simulink model "ess_balancing_rig"  (R2025b)
settings: Solver=ode23t  StartTime=0.0  StopTime=10800  MaxStep=1  RelTol=1e-3
PreLoadFcn:
  | I_chg   = 1.25;               % charge current [A] (0.5C)
  | R_bleed = 47;                 % balancing (bleed) resistor [Ohm]
  | SOC0    = [0.80 0.75 0.75];   % initial SOC of Cell, Cell1, Cell2
libraries: nesl_utility x18, fl_lib x16, batteryecm_lib x3, BatteryBalancing x1
settings Model: Creator=Saquire  LastModifiedBy=Saquire
settings DataIOCC: SaveOutput=off

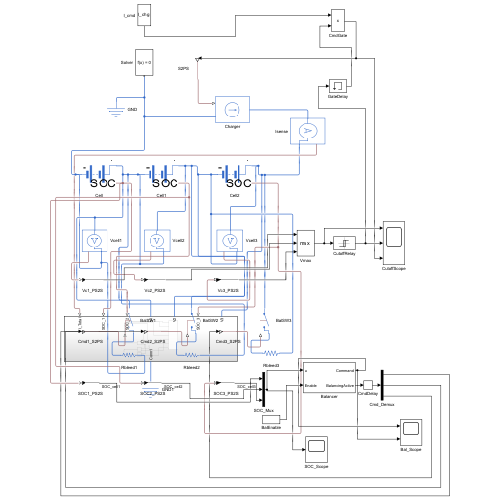
[thumbnail: Simulink's stored preview of the top-level diagram]
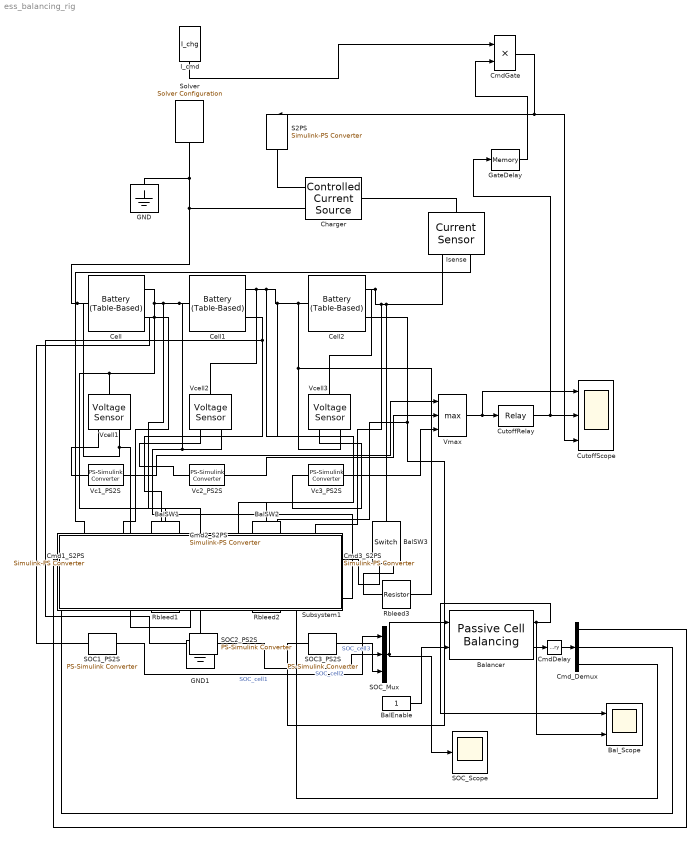
== system ess_balancing_rig ==
  BalEnable : Constant  OutDataTypeStr=boolean
  BalSW1 : fl_lib/Electrical/Electrical Elements/Switch  R_closed=0.01 Ohm  G_open=1e-8 1/Ohm  Threshold=0.5  i_specify=off  i_priority=None  i=0 A  i_nominal_specify=off  i_nominal_value=1  i_nominal_unit=A  v_specify=off  v_priority=None  v=0 V  v_nominal_specify=off  v_nominal_value=1  v_nominal_unit=V
  BalSW2 : fl_lib/Electrical/Electrical Elements/Switch  R_closed=0.01 Ohm  G_open=1e-8 1/Ohm  Threshold=0.5  i_specify=off  i_priority=None  i=0 A  i_nominal_specify=off  i_nominal_value=1  i_nominal_unit=A  v_specify=off  v_priority=None  v=0 V  v_nominal_specify=off  v_nominal_value=1  v_nominal_unit=V
  BalSW3 : fl_lib/Electrical/Electrical Elements/Switch  R_closed=0.01 Ohm  G_open=1e-8 1/Ohm  Threshold=0.5  i_specify=off  i_priority=None  i=0 A  i_nominal_specify=off  i_nominal_value=1  i_nominal_unit=A  v_specify=off  v_priority=None  v=0 V  v_nominal_specify=off  v_nominal_value=1  v_nominal_unit=V
  Bal_Scope : Scope  NumInputPorts=2
      settings: Title=Balancing commands / active  DataLoggingVariableName=balData
  Balancer : BatteryBalancing/Passive Cell Balancing  Threshold=0.01  HysteresisBand=0.005  Td_on=1  Td_off=1  Ts=1  dataType=double
      settings: LibrarySourceBlock=batt_sl_lib/Cell Balancing/Passive Cell Balancing
  Cell : batteryecm_lib/Battery (Table-Based)  SOC_vec=[0 .1 .2 .3 .4 .5 .6 .7 .8 .9 1]  T_dependence=simscape.enum.tablebattery.temperature_dependence.yes  prm_dir=simscape.enum.tablebattery.prm_dir.noCurrentDirectionality  T_vec=[278 293 313] K  V0_mat=[3.00 3.05 3.08;3.42 3.45 3.47;3.53 3.55 3.57;3.60 3.62 3.64;3.65 3.67 3.69;3.70 3.72 3.74;3.78 3.80 3.82;3.88 3.90 3.92;3.97 3.99 4.01;4.06 4.08 4.10;4.16 4.18 4.19] V  V0_vec=[3.5057, 3.566, 3.6337, 3.7127, 3.9259, 4.0777, 4.1928] V  V_range=[2.5 4.3] V  R0_mat=[.070 .045 .035;.055 .036 .028;.050 .033 .026;.048 .032 .025;.046 .031 .024;.045 .030 .024;.045 .030 .024;.045 .030 .024;.046 .031 .025;.047 .031 .025;.048 .032 .026] Ohm  R0_vec=[.0085, .0085, .0087, .0082, .0083, .0085, .0085] Ohm  R0_dis_mat=[.0117, .0085, .009; .011, .0085, .009; .0114, .0087, .0092; .0107, .0082, .0088; .0107, .0083, .0091; .0113, .0085, .0089; .0116, .0085, .0089] Ohm  R0_dis_vec=[.0085, .0085, .0087, .0082, .0083, .0085, .0085] Ohm  R0_ch_mat=[.0117, .0085, .009; .011, .0085, .009; .0114, .0087, .0092; .0107, .0082, .0088; .0107, .0083, .0091; .0113, .0085, .0089; .0116, .0085, .0089] Ohm  R0_ch_vec=[.0085, .0085, .0087, .0082, .0083, .0085, .0085] Ohm  AH=2.5 A*hr  prm_leak=simscape.enum.tablebattery.prm_leak.disabled  Rleak_vec=[8000, 7000, 6000] Ohm  Rleak=7e3 Ohm  extrapolation_option=simscape.enum.extrapolation.nearest  SOC_port=simscape.enum.tablebattery.enable.yes  prm_dyn=simscape.enum.tablebattery.prm_dyn.off  R1_mat=[.0109, .0029, .0013; .0069, .0024, .0012; .0047, .0026, .0013; .0034, .0016, .001; .0033, .0023, .0014; .0033, .0018, .0011; .0028, .0017, .0011] Ohm  R1_vec=[.0029, .0024, .0026, .0016, .0023, .0018, .0017] Ohm  tau1_mat=[20, 36, 39; 31, 45, 39; 109, 105, 61; 36, 29, 26; 59, 77, 67; 40, 33, 29; 25, 39, 33] s  tau1_vec=[36, 45, 105, 29, 77, 33, 39] s  R2_mat=[.0109, .0029, .0013; .0069, .0024, .0012; .0047, .0026, .0013; .0034, .0016, .001; .0033, .0023, .0014; .0033, .0018, .0011; .0028, .0017, .0011] Ohm  R2_vec=[.0029, .0024, .0026, .0016, .0023, .0018, .0017] Ohm  tau2_mat=[20, 36, 39; 31, 45, 39; 109, 105, 61; 36, 29, 26; 59, 77, 67; 40, 33, 29; 25, 39, 33] s  tau2_vec=[36, 45, 105, 29, 77, 33, 39] s  R3_mat=[.0109, .0029, .0013; .0069, .0024, .0012; .0047, .0026, .0013; .0034, .0016, .001; .0033, .0023, .0014; .0033, .0018, .0011; .0028, .0017, .0011] Ohm  R3_vec=[.0029, .0024, .0026, .0016, .0023, .0018, .0017] Ohm  tau3_mat=[20, 36, 39; 31, 45, 39; 109, 105, 61; 36, 29, 26; 59, 77, 67; 40, 33, 29; 25, 39, 33] s  tau3_vec=[36, 45, 105, 29, 77, 33, 39] s  R4_mat=[.0109, .0029, .0013; .0069, .0024, .0012; .0047, .0026, .0013; .0034, .0016, .001; .0033, .0023, .0014; .0033, .0018, .0011; .0028, .0017, .0011] Ohm  R4_vec=[.0029, .0024, .0026, .0016, .0023, .0018, .0017] Ohm  tau4_mat=[20, 36, 39; 31, 45, 39; 109, 105, 61; 36, 29, 26; 59, 77, 67; 40, 33, 29; 25, 39, 33] s  tau4_vec=[36, 45, 105, 29, 77, 33, 39] s  R5_mat=[.0109, .0029, .0013; .0069, .0024, .0012; .0047, .0026, .0013; .0034, .0016, .001; .0033, .0023, .0014; .0033, .0018, .0011; .0028, .0017, .0011] Ohm  R5_vec=[.0029, .0024, .0026, .0016, .0023, .0018, .0017] Ohm  tau5_mat=[20, 36, 39; 31, 45, 39; 109, 105, 61; 36, 29, 26; 59, 77, 67; 40, 33, 29; 25, 39, 33] s  tau5_vec=[36, 45, 105, 29, 77, 33, 39] s  prm_fade=simscape.enum.tablebattery.prm_fade.disabled  N0=100  dV0=0  dR0=0  dAH=0  dRleak=0  dR1=0  dR2=0  dR3=0  dR4=0  dR5=0  N0vec=[0, 100, 200, 300]  Tfadevec=[298.15, 323.15] K  dV0vec=[0, 0, 0, 0]  dR0vec=[0, 0, 0, 0]  dAHvec=[0, 0, 0, 0]  dRleakvec=[0, 0, 0, 0]  dR1vec=[0, 0, 0, 0]  dR2vec=[0, 0, 0, 0]  dR3vec=[0, 0, 0, 0]  dR4vec=[0, 0, 0, 0]  dR5vec=[0, 0, 0, 0]  dV0mat=[0, 0; 0, 0; 0, 0; 0, 0]  dR0mat=[0, 0; 0, 0; 0, 0; 0, 0]  dAHmat=[0, 0; 0, 0; 0, 0; 0, 0]  dRleakmat=[0, 0; 0, 0; 0, 0; 0, 0]  dR1mat=[0, 0; 0, 0; 0, 0; 0, 0]  dR2mat=[0, 0; 0, 0; 0, 0; 0, 0]  dR3mat=[0, 0; 0, 0; 0, 0; 0, 0]  dR4mat=[0, 0; 0, 0; 0, 0; 0, 0]  dR5mat=[0, 0; 0, 0; 0, 0; 0, 0]  prm_age_modeling=simscape.enum.tablebattery.prm_age_modeling.equation  storage_dt_age_vec=[0] d  storage_T_age_vec=[273] K  prm_age_OCV=simscape.enum.tablebattery.prm_age_OCV.OCV  OCV_age=0.9  SOC_age=0.6  prm_age_resistance=simscape.enum.tablebattery.prm_age.disabled  OCV_scaling_age_resistance=2.2134e6  OCV_offset_age_resistance=1.632e6  temp_exp_age_resistance=0.515833569 V  t_exp_age_resistance=0.75  T_age_vec_resistance=[273.15, 298.15, 323.15] K  dt_age_vec_resistance=[0, 90, 180, 270] d  dR0_age_vec=[0, 0, 0]  t_meas_dR0_age=100 d  dR0_age_mat=[0, 0, 0; 0, 0, 0; 0, 0, 0; 0, 0, 0]  prm_age_capacity=simscape.enum.tablebattery.prm_age.disabled  OCV_scaling_age_capacity=1.5097e07  OCV_offset_age_capacity=8.3625e06  temp_exp_age_capacity=0.6011 V  t_exp_age_capacity=0.75  T_age_vec_capacity=[273.15, 298.15, 323.15] K  dt_age_vec_capacity=[0, 90, 180, 270] d  dAH_age_vec=[0, 0, 0]  t_meas_dAH_age=100 d  dAH_age_mat=[0, 0, 0; 0, 0, 0; 0, 0, 0; 0, 0, 0]  thermal_port=simscape.enum.thermaleffects.omit  temperature=298.15 K  thermal_mass=100 J/K  i_specify=off  i_priority=None  i=0 A  i_nominal_specify=off  i_nominal_value=1  i_nominal_unit=A  v_specify=off  v_priority=None  v=0 V  v_nominal_specify=off  v_nominal_value=1  v_nominal_unit=V  stateOfCharge_specify=on  stateOfCharge_priority=High  stateOfCharge=SOC0(1)  stateOfCharge_nominal_specify=off  stateOfCharge_nominal_value=1  stateOfCharge_nominal_unit=1  num_cycles_specify=off  num_cycles_priority=High  num_cycles=0  num_cycles_nominal_specify=off  num_cycles_nominal_value=1  num_cycles_nominal_unit=1  cell_temperature_specify=off  cell_temperature_priority=High  cell_temperature=298.15 K  cell_temperature_nominal_specify=off  cell_temperature_nominal_value=1  cell_temperature_nominal_unit=K
      settings: InternalSimscapePortConfiguration="{\"Bottom\":[],\"Left\":[{\"id\":\"p\",\"label\":\"+\",\"type\":\"foundation.electrical.electrical\"},{\"id\":\"soc\",\"label\":\"SOC\",\"type\":\"output\"}],\"Right\":[{\"id\":\"n\",\"label\":\"-\",\"type\":\"foundation.electrical.electrical\"}],\"Top\":[]}"
  Cell1 : batteryecm_lib/Battery (Table-Based)  SOC_vec=[0 .1 .2 .3 .4 .5 .6 .7 .8 .9 1]  T_dependence=simscape.enum.tablebattery.temperature_dependence.yes  prm_dir=simscape.enum.tablebattery.prm_dir.noCurrentDirectionality  T_vec=[278 293 313] K  V0_mat=[3.00 3.05 3.08;3.42 3.45 3.47;3.53 3.55 3.57;3.60 3.62 3.64;3.65 3.67 3.69;3.70 3.72 3.74;3.78 3.80 3.82;3.88 3.90 3.92;3.97 3.99 4.01;4.06 4.08 4.10;4.16 4.18 4.19] V  V0_vec=[3.5057, 3.566, 3.6337, 3.7127, 3.9259, 4.0777, 4.1928] V  V_range=[2.5 4.3] V  R0_mat=[.070 .045 .035;.055 .036 .028;.050 .033 .026;.048 .032 .025;.046 .031 .024;.045 .030 .024;.045 .030 .024;.045 .030 .024;.046 .031 .025;.047 .031 .025;.048 .032 .026] Ohm  R0_vec=[.0085, .0085, .0087, .0082, .0083, .0085, .0085] Ohm  R0_dis_mat=[.0117, .0085, .009; .011, .0085, .009; .0114, .0087, .0092; .0107, .0082, .0088; .0107, .0083, .0091; .0113, .0085, .0089; .0116, .0085, .0089] Ohm  R0_dis_vec=[.0085, .0085, .0087, .0082, .0083, .0085, .0085] Ohm  R0_ch_mat=[.0117, .0085, .009; .011, .0085, .009; .0114, .0087, .0092; .0107, .0082, .0088; .0107, .0083, .0091; .0113, .0085, .0089; .0116, .0085, .0089] Ohm  R0_ch_vec=[.0085, .0085, .0087, .0082, .0083, .0085, .0085] Ohm  AH=2.5 A*hr  prm_leak=simscape.enum.tablebattery.prm_leak.disabled  Rleak_vec=[8000, 7000, 6000] Ohm  Rleak=7e3 Ohm  extrapolation_option=simscape.enum.extrapolation.nearest  SOC_port=simscape.enum.tablebattery.enable.yes  prm_dyn=simscape.enum.tablebattery.prm_dyn.off  R1_mat=[.0109, .0029, .0013; .0069, .0024, .0012; .0047, .0026, .0013; .0034, .0016, .001; .0033, .0023, .0014; .0033, .0018, .0011; .0028, .0017, .0011] Ohm  R1_vec=[.0029, .0024, .0026, .0016, .0023, .0018, .0017] Ohm  tau1_mat=[20, 36, 39; 31, 45, 39; 109, 105, 61; 36, 29, 26; 59, 77, 67; 40, 33, 29; 25, 39, 33] s  tau1_vec=[36, 45, 105, 29, 77, 33, 39] s  R2_mat=[.0109, .0029, .0013; .0069, .0024, .0012; .0047, .0026, .0013; .0034, .0016, .001; .0033, .0023, .0014; .0033, .0018, .0011; .0028, .0017, .0011] Ohm  R2_vec=[.0029, .0024, .0026, .0016, .0023, .0018, .0017] Ohm  tau2_mat=[20, 36, 39; 31, 45, 39; 109, 105, 61; 36, 29, 26; 59, 77, 67; 40, 33, 29; 25, 39, 33] s  tau2_vec=[36, 45, 105, 29, 77, 33, 39] s  R3_mat=[.0109, .0029, .0013; .0069, .0024, .0012; .0047, .0026, .0013; .0034, .0016, .001; .0033, .0023, .0014; .0033, .0018, .0011; .0028, .0017, .0011] Ohm  R3_vec=[.0029, .0024, .0026, .0016, .0023, .0018, .0017] Ohm  tau3_mat=[20, 36, 39; 31, 45, 39; 109, 105, 61; 36, 29, 26; 59, 77, 67; 40, 33, 29; 25, 39, 33] s  tau3_vec=[36, 45, 105, 29, 77, 33, 39] s  R4_mat=[.0109, .0029, .0013; .0069, .0024, .0012; .0047, .0026, .0013; .0034, .0016, .001; .0033, .0023, .0014; .0033, .0018, .0011; .0028, .0017, .0011] Ohm  R4_vec=[.0029, .0024, .0026, .0016, .0023, .0018, .0017] Ohm  tau4_mat=[20, 36, 39; 31, 45, 39; 109, 105, 61; 36, 29, 26; 59, 77, 67; 40, 33, 29; 25, 39, 33] s  tau4_vec=[36, 45, 105, 29, 77, 33, 39] s  R5_mat=[.0109, .0029, .0013; .0069, .0024, .0012; .0047, .0026, .0013; .0034, .0016, .001; .0033, .0023, .0014; .0033, .0018, .0011; .0028, .0017, .0011] Ohm  R5_vec=[.0029, .0024, .0026, .0016, .0023, .0018, .0017] Ohm  tau5_mat=[20, 36, 39; 31, 45, 39; 109, 105, 61; 36, 29, 26; 59, 77, 67; 40, 33, 29; 25, 39, 33] s  tau5_vec=[36, 45, 105, 29, 77, 33, 39] s  prm_fade=simscape.enum.tablebattery.prm_fade.disabled  N0=100  dV0=0  dR0=0  dAH=0  dRleak=0  dR1=0  dR2=0  dR3=0  dR4=0  dR5=0  N0vec=[0, 100, 200, 300]  Tfadevec=[298.15, 323.15] K  dV0vec=[0, 0, 0, 0]  dR0vec=[0, 0, 0, 0]  dAHvec=[0, 0, 0, 0]  dRleakvec=[0, 0, 0, 0]  dR1vec=[0, 0, 0, 0]  dR2vec=[0, 0, 0, 0]  dR3vec=[0, 0, 0, 0]  dR4vec=[0, 0, 0, 0]  dR5vec=[0, 0, 0, 0]  dV0mat=[0, 0; 0, 0; 0, 0; 0, 0]  dR0mat=[0, 0; 0, 0; 0, 0; 0, 0]  dAHmat=[0, 0; 0, 0; 0, 0; 0, 0]  dRleakmat=[0, 0; 0, 0; 0, 0; 0, 0]  dR1mat=[0, 0; 0, 0; 0, 0; 0, 0]  dR2mat=[0, 0; 0, 0; 0, 0; 0, 0]  dR3mat=[0, 0; 0, 0; 0, 0; 0, 0]  dR4mat=[0, 0; 0, 0; 0, 0; 0, 0]  dR5mat=[0, 0; 0, 0; 0, 0; 0, 0]  prm_age_modeling=simscape.enum.tablebattery.prm_age_modeling.equation  storage_dt_age_vec=[0] d  storage_T_age_vec=[273] K  prm_age_OCV=simscape.enum.tablebattery.prm_age_OCV.OCV  OCV_age=0.9  SOC_age=0.6  prm_age_resistance=simscape.enum.tablebattery.prm_age.disabled  OCV_scaling_age_resistance=2.2134e6  OCV_offset_age_resistance=1.632e6  temp_exp_age_resistance=0.515833569 V  t_exp_age_resistance=0.75  T_age_vec_resistance=[273.15, 298.15, 323.15] K  dt_age_vec_resistance=[0, 90, 180, 270] d  dR0_age_vec=[0, 0, 0]  t_meas_dR0_age=100 d  dR0_age_mat=[0, 0, 0; 0, 0, 0; 0, 0, 0; 0, 0, 0]  prm_age_capacity=simscape.enum.tablebattery.prm_age.disabled  OCV_scaling_age_capacity=1.5097e07  OCV_offset_age_capacity=8.3625e06  temp_exp_age_capacity=0.6011 V  t_exp_age_capacity=0.75  T_age_vec_capacity=[273.15, 298.15, 323.15] K  dt_age_vec_capacity=[0, 90, 180, 270] d  dAH_age_vec=[0, 0, 0]  t_meas_dAH_age=100 d  dAH_age_mat=[0, 0, 0; 0, 0, 0; 0, 0, 0; 0, 0, 0]  thermal_port=simscape.enum.thermaleffects.omit  temperature=298.15 K  thermal_mass=100 J/K  i_specify=off  i_priority=None  i=0 A  i_nominal_specify=off  i_nominal_value=1  i_nominal_unit=A  v_specify=off  v_priority=None  v=0 V  v_nominal_specify=off  v_nominal_value=1  v_nominal_unit=V  stateOfCharge_specify=on  stateOfCharge_priority=High  stateOfCharge=SOC0(2)  stateOfCharge_nominal_specify=off  stateOfCharge_nominal_value=0.6  stateOfCharge_nominal_unit=1  num_cycles_specify=off  num_cycles_priority=High  num_cycles=0  num_cycles_nominal_specify=off  num_cycles_nominal_value=1  num_cycles_nominal_unit=1  cell_temperature_specify=off  cell_temperature_priority=High  cell_temperature=298.15 K  cell_temperature_nominal_specify=off  cell_temperature_nominal_value=1  cell_temperature_nominal_unit=K
      settings: InternalSimscapePortConfiguration="{\"Bottom\":[],\"Left\":[{\"id\":\"p\",\"label\":\"+\",\"type\":\"foundation.electrical.electrical\"},{\"id\":\"soc\",\"label\":\"SOC\",\"type\":\"output\"}],\"Right\":[{\"id\":\"n\",\"label\":\"-\",\"type\":\"foundation.electrical.electrical\"}],\"Top\":[]}"
  Cell2 : batteryecm_lib/Battery (Table-Based)  SOC_vec=[0 .1 .2 .3 .4 .5 .6 .7 .8 .9 1]  T_dependence=simscape.enum.tablebattery.temperature_dependence.yes  prm_dir=simscape.enum.tablebattery.prm_dir.noCurrentDirectionality  T_vec=[278 293 313] K  V0_mat=[3.00 3.05 3.08;3.42 3.45 3.47;3.53 3.55 3.57;3.60 3.62 3.64;3.65 3.67 3.69;3.70 3.72 3.74;3.78 3.80 3.82;3.88 3.90 3.92;3.97 3.99 4.01;4.06 4.08 4.10;4.16 4.18 4.19] V  V0_vec=[3.5057, 3.566, 3.6337, 3.7127, 3.9259, 4.0777, 4.1928] V  V_range=[2.5 4.3] V  R0_mat=[.070 .045 .035;.055 .036 .028;.050 .033 .026;.048 .032 .025;.046 .031 .024;.045 .030 .024;.045 .030 .024;.045 .030 .024;.046 .031 .025;.047 .031 .025;.048 .032 .026] Ohm  R0_vec=[.0085, .0085, .0087, .0082, .0083, .0085, .0085] Ohm  R0_dis_mat=[.0117, .0085, .009; .011, .0085, .009; .0114, .0087, .0092; .0107, .0082, .0088; .0107, .0083, .0091; .0113, .0085, .0089; .0116, .0085, .0089] Ohm  R0_dis_vec=[.0085, .0085, .0087, .0082, .0083, .0085, .0085] Ohm  R0_ch_mat=[.0117, .0085, .009; .011, .0085, .009; .0114, .0087, .0092; .0107, .0082, .0088; .0107, .0083, .0091; .0113, .0085, .0089; .0116, .0085, .0089] Ohm  R0_ch_vec=[.0085, .0085, .0087, .0082, .0083, .0085, .0085] Ohm  AH=2.5 A*hr  prm_leak=simscape.enum.tablebattery.prm_leak.disabled  Rleak_vec=[8000, 7000, 6000] Ohm  Rleak=7e3 Ohm  extrapolation_option=simscape.enum.extrapolation.nearest  SOC_port=simscape.enum.tablebattery.enable.yes  prm_dyn=simscape.enum.tablebattery.prm_dyn.off  R1_mat=[.0109, .0029, .0013; .0069, .0024, .0012; .0047, .0026, .0013; .0034, .0016, .001; .0033, .0023, .0014; .0033, .0018, .0011; .0028, .0017, .0011] Ohm  R1_vec=[.0029, .0024, .0026, .0016, .0023, .0018, .0017] Ohm  tau1_mat=[20, 36, 39; 31, 45, 39; 109, 105, 61; 36, 29, 26; 59, 77, 67; 40, 33, 29; 25, 39, 33] s  tau1_vec=[36, 45, 105, 29, 77, 33, 39] s  R2_mat=[.0109, .0029, .0013; .0069, .0024, .0012; .0047, .0026, .0013; .0034, .0016, .001; .0033, .0023, .0014; .0033, .0018, .0011; .0028, .0017, .0011] Ohm  R2_vec=[.0029, .0024, .0026, .0016, .0023, .0018, .0017] Ohm  tau2_mat=[20, 36, 39; 31, 45, 39; 109, 105, 61; 36, 29, 26; 59, 77, 67; 40, 33, 29; 25, 39, 33] s  tau2_vec=[36, 45, 105, 29, 77, 33, 39] s  R3_mat=[.0109, .0029, .0013; .0069, .0024, .0012; .0047, .0026, .0013; .0034, .0016, .001; .0033, .0023, .0014; .0033, .0018, .0011; .0028, .0017, .0011] Ohm  R3_vec=[.0029, .0024, .0026, .0016, .0023, .0018, .0017] Ohm  tau3_mat=[20, 36, 39; 31, 45, 39; 109, 105, 61; 36, 29, 26; 59, 77, 67; 40, 33, 29; 25, 39, 33] s  tau3_vec=[36, 45, 105, 29, 77, 33, 39] s  R4_mat=[.0109, .0029, .0013; .0069, .0024, .0012; .0047, .0026, .0013; .0034, .0016, .001; .0033, .0023, .0014; .0033, .0018, .0011; .0028, .0017, .0011] Ohm  R4_vec=[.0029, .0024, .0026, .0016, .0023, .0018, .0017] Ohm  tau4_mat=[20, 36, 39; 31, 45, 39; 109, 105, 61; 36, 29, 26; 59, 77, 67; 40, 33, 29; 25, 39, 33] s  tau4_vec=[36, 45, 105, 29, 77, 33, 39] s  R5_mat=[.0109, .0029, .0013; .0069, .0024, .0012; .0047, .0026, .0013; .0034, .0016, .001; .0033, .0023, .0014; .0033, .0018, .0011; .0028, .0017, .0011] Ohm  R5_vec=[.0029, .0024, .0026, .0016, .0023, .0018, .0017] Ohm  tau5_mat=[20, 36, 39; 31, 45, 39; 109, 105, 61; 36, 29, 26; 59, 77, 67; 40, 33, 29; 25, 39, 33] s  tau5_vec=[36, 45, 105, 29, 77, 33, 39] s  prm_fade=simscape.enum.tablebattery.prm_fade.disabled  N0=100  dV0=0  dR0=0  dAH=0  dRleak=0  dR1=0  dR2=0  dR3=0  dR4=0  dR5=0  N0vec=[0, 100, 200, 300]  Tfadevec=[298.15, 323.15] K  dV0vec=[0, 0, 0, 0]  dR0vec=[0, 0, 0, 0]  dAHvec=[0, 0, 0, 0]  dRleakvec=[0, 0, 0, 0]  dR1vec=[0, 0, 0, 0]  dR2vec=[0, 0, 0, 0]  dR3vec=[0, 0, 0, 0]  dR4vec=[0, 0, 0, 0]  dR5vec=[0, 0, 0, 0]  dV0mat=[0, 0; 0, 0; 0, 0; 0, 0]  dR0mat=[0, 0; 0, 0; 0, 0; 0, 0]  dAHmat=[0, 0; 0, 0; 0, 0; 0, 0]  dRleakmat=[0, 0; 0, 0; 0, 0; 0, 0]  dR1mat=[0, 0; 0, 0; 0, 0; 0, 0]  dR2mat=[0, 0; 0, 0; 0, 0; 0, 0]  dR3mat=[0, 0; 0, 0; 0, 0; 0, 0]  dR4mat=[0, 0; 0, 0; 0, 0; 0, 0]  dR5mat=[0, 0; 0, 0; 0, 0; 0, 0]  prm_age_modeling=simscape.enum.tablebattery.prm_age_modeling.equation  storage_dt_age_vec=[0] d  storage_T_age_vec=[273] K  prm_age_OCV=simscape.enum.tablebattery.prm_age_OCV.OCV  OCV_age=0.9  SOC_age=0.6  prm_age_resistance=simscape.enum.tablebattery.prm_age.disabled  OCV_scaling_age_resistance=2.2134e6  OCV_offset_age_resistance=1.632e6  temp_exp_age_resistance=0.515833569 V  t_exp_age_resistance=0.75  T_age_vec_resistance=[273.15, 298.15, 323.15] K  dt_age_vec_resistance=[0, 90, 180, 270] d  dR0_age_vec=[0, 0, 0]  t_meas_dR0_age=100 d  dR0_age_mat=[0, 0, 0; 0, 0, 0; 0, 0, 0; 0, 0, 0]  prm_age_capacity=simscape.enum.tablebattery.prm_age.disabled  OCV_scaling_age_capacity=1.5097e07  OCV_offset_age_capacity=8.3625e06  temp_exp_age_capacity=0.6011 V  t_exp_age_capacity=0.75  T_age_vec_capacity=[273.15, 298.15, 323.15] K  dt_age_vec_capacity=[0, 90, 180, 270] d  dAH_age_vec=[0, 0, 0]  t_meas_dAH_age=100 d  dAH_age_mat=[0, 0, 0; 0, 0, 0; 0, 0, 0; 0, 0, 0]  thermal_port=simscape.enum.thermaleffects.omit  temperature=298.15 K  thermal_mass=100 J/K  i_specify=off  i_priority=None  i=0 A  i_nominal_specify=off  i_nominal_value=1  i_nominal_unit=A  v_specify=off  v_priority=None  v=0 V  v_nominal_specify=off  v_nominal_value=1  v_nominal_unit=V  stateOfCharge_specify=on  stateOfCharge_priority=High  stateOfCharge=SOC0(3)  stateOfCharge_nominal_specify=off  stateOfCharge_nominal_value=0.6  stateOfCharge_nominal_unit=1  num_cycles_specify=off  num_cycles_priority=High  num_cycles=0  num_cycles_nominal_specify=off  num_cycles_nominal_value=1  num_cycles_nominal_unit=1  cell_temperature_specify=off  cell_temperature_priority=High  cell_temperature=298.15 K  cell_temperature_nominal_specify=off  cell_temperature_nominal_value=1  cell_temperature_nominal_unit=K
      settings: InternalSimscapePortConfiguration="{\"Bottom\":[],\"Left\":[{\"id\":\"p\",\"label\":\"+\",\"type\":\"foundation.electrical.electrical\"},{\"id\":\"soc\",\"label\":\"SOC\",\"type\":\"output\"}],\"Right\":[{\"id\":\"n\",\"label\":\"-\",\"type\":\"foundation.electrical.electrical\"}],\"Top\":[]}"
  Charger : fl_lib/Electrical/Electrical Sources/Controlled Current Source
  Cmd1_S2PS : nesl_utility/Simulink-PS Converter  PhysicalDomain=network_engine_domain  SubClassName=ps_input  LeftPortType=input  RightPortType=output  PseudoPeriodic=off  Frequencies=[]  NoiseDistribution=none  NoiseParameters=[]  Unit=1  AffineConversion=off  FilteringAndDerivatives=provide  SimscapeFilterOrder=1  InputFilterTimeConstant=0.001  UdotUserProvided=0
  Cmd2_S2PS : nesl_utility/Simulink-PS Converter  PhysicalDomain=network_engine_domain  SubClassName=ps_input  LeftPortType=input  RightPortType=output  PseudoPeriodic=off  Frequencies=[]  NoiseDistribution=none  NoiseParameters=[]  Unit=1  AffineConversion=off  FilteringAndDerivatives=provide  SimscapeFilterOrder=1  InputFilterTimeConstant=0.001  UdotUserProvided=0
  Cmd3_S2PS : nesl_utility/Simulink-PS Converter  PhysicalDomain=network_engine_domain  SubClassName=ps_input  LeftPortType=input  RightPortType=output  PseudoPeriodic=off  Frequencies=[]  NoiseDistribution=none  NoiseParameters=[]  Unit=1  AffineConversion=off  FilteringAndDerivatives=provide  SimscapeFilterOrder=1  InputFilterTimeConstant=0.001  UdotUserProvided=0
  CmdDelay : Memory
  CmdGate : Product
  Cmd_Demux : Demux  Outputs=3
  CutoffRelay : Relay  OnSwitchValue=4.2  OffSwitchValue=4.15  OnOutputValue=0  OffOutputValue=1
  CutoffScope : Scope  NumInputPorts=3
      settings: ActiveDisplayYMinimum=-9.1766114496806388  ActiveDisplayYMaximum=10.823388550319361  DataLoggingVariableName=cutoffData
  GND : fl_lib/Electrical/Electrical Elements/Electrical Reference
  GND1 : fl_lib/Electrical/Electrical Elements/Electrical Reference
  GateDelay : Memory  InitialCondition=1
  I_cmd : Constant  Value=I_chg
  Isense : fl_lib/Electrical/Electrical Sensors/Current Sensor
  Rbleed1 : fl_lib/Electrical/Electrical Elements/Resistor  R=R_bleed Ohm  i_specify=off  i_priority=None  i=0 A  i_nominal_specify=off  i_nominal_value=1  i_nominal_unit=A  v_specify=off  v_priority=None  v=0 V  v_nominal_specify=off  v_nominal_value=1  v_nominal_unit=V
  Rbleed2 : fl_lib/Electrical/Electrical Elements/Resistor  R=R_bleed Ohm  i_specify=off  i_priority=None  i=0 A  i_nominal_specify=off  i_nominal_value=1  i_nominal_unit=A  v_specify=off  v_priority=None  v=0 V  v_nominal_specify=off  v_nominal_value=1  v_nominal_unit=V
  Rbleed3 : fl_lib/Electrical/Electrical Elements/Resistor  R=R_bleed Ohm  i_specify=off  i_priority=None  i=0 A  i_nominal_specify=off  i_nominal_value=1  i_nominal_unit=A  v_specify=off  v_priority=None  v=0 V  v_nominal_specify=off  v_nominal_value=1  v_nominal_unit=V
  S2PS : nesl_utility/Simulink-PS Converter  PhysicalDomain=network_engine_domain  SubClassName=ps_input  LeftPortType=input  RightPortType=output  PseudoPeriodic=off  Frequencies=[]  NoiseDistribution=none  NoiseParameters=[]  Unit=1  AffineConversion=off  FilteringAndDerivatives=provide  SimscapeFilterOrder=1  InputFilterTimeConstant=0.001  UdotUserProvided=0
  SOC1_PS2S : nesl_utility/PS-Simulink Converter  PhysicalDomain=network_engine_domain  SubClassName=ps_output  LeftPortType=input  RightPortType=output  PseudoPeriodic=off  Frequencies=[]  VectorFormat=inherit  Unit=inherit  AffineConversion=off
  SOC2_PS2S : nesl_utility/PS-Simulink Converter  PhysicalDomain=network_engine_domain  SubClassName=ps_output  LeftPortType=input  RightPortType=output  PseudoPeriodic=off  Frequencies=[]  VectorFormat=inherit  Unit=inherit  AffineConversion=off
  SOC3_PS2S : nesl_utility/PS-Simulink Converter  PhysicalDomain=network_engine_domain  SubClassName=ps_output  LeftPortType=input  RightPortType=output  PseudoPeriodic=off  Frequencies=[]  VectorFormat=inherit  Unit=inherit  AffineConversion=off
  SOC_Mux : Mux  Inputs=3
  SOC_Scope : Scope
      settings: Title=Cell SOCs  ActiveDisplayYMinimum=0.7  ActiveDisplayYMaximum=1  YLabel=SOC  DataLoggingVariableName=socData
  Solver : nesl_utility/Solver Configuration  PhysicalDomain=network_engine_domain  SubClassName=solver  LeftPortType=input  RightPortType=generic  Tones=[]  Harmonics=[]  SimulateNoise=off  Profile=off  UseLocalSampling=off  EnableSwitchedLinearOptims=on  FrequencyDomain=off  UseCCode=off  RelTol=0.001  AbsTol=0.001  MinStep=1e-09  ToWorkspace=off  RevertToSquareIcSolve=off  NumHomotopyIterations=100  PhasorMode=off  PhasorModeNumHarmonics=1  ConsistencySolver=NEWTON_XTOL_AFTER_FTOL  IndexReductionMethod=DerivativeReplacement  DoDC=off  ResidualTolerance=1e-09  ConsistencyTolSource=GLOBAL  ConsistencyAbsTol=0.001  ConsistencyRelTol=0.001  ConsistencyTolFactor=0.001  UseLocalSolver=off  LocalSolverChoice=NE_BACKWARD_EULER_ADVANCER  ResolveIndetEquations=on  FunctionEvalNumThread=1  LocalSolverSampleTime=0.001  DoFixedCost=off  MaxNonlinIter=3  MaxModeIter=2  ComputeImpulses=off  ImpulseIterations=2  LinearAlgebra=auto  LinearAlgebraNumThread=0  EquationFormulation=NE_TIME_EF  DelaysMemoryBudget=1024  AutomaticFiltering=on  FilteringTimeConstant=0.001  PartitionStorageMethod=AS_NEEDED  PartitionMemoryBudget=1024  PartitionMethod=ROBUST  MultibodyUseLocalSolver=off  MultibodyLocalSolverChoice=ODE1  MultibodyLocalSolverSampleTime=0.001
  Subsystem1 : Subsystem
  Vc1_PS2S : nesl_utility/PS-Simulink Converter  PhysicalDomain=network_engine_domain  SubClassName=ps_output  LeftPortType=input  RightPortType=output  PseudoPeriodic=off  Frequencies=[]  VectorFormat=inherit  Unit=inherit  AffineConversion=off
  Vc2_PS2S : nesl_utility/PS-Simulink Converter  PhysicalDomain=network_engine_domain  SubClassName=ps_output  LeftPortType=input  RightPortType=output  PseudoPeriodic=off  Frequencies=[]  VectorFormat=inherit  Unit=inherit  AffineConversion=off
  Vc3_PS2S : nesl_utility/PS-Simulink Converter  PhysicalDomain=network_engine_domain  SubClassName=ps_output  LeftPortType=input  RightPortType=output  PseudoPeriodic=off  Frequencies=[]  VectorFormat=inherit  Unit=inherit  AffineConversion=off
  Vcell1 : fl_lib/Electrical/Electrical Sensors/Voltage Sensor
  Vcell2 : fl_lib/Electrical/Electrical Sensors/Voltage Sensor
  Vcell3 : fl_lib/Electrical/Electrical Sensors/Voltage Sensor
  Vmax : MinMax  Function=max  Inputs=3
  wires:
  Vc1_PS2S/1 -> Vmax/1
  Vc2_PS2S/1 -> Vmax/2
  Vc3_PS2S/1 -> Vmax/3
  Vmax/1 -> CutoffRelay/1, CutoffScope/1
  I_cmd/1 -> CmdGate/1
  CutoffRelay/1 -> CutoffScope/2, GateDelay/1
  CmdGate/1 -> S2PS/1, CutoffScope/3
  GateDelay/1 -> CmdGate/2
  SOC1_PS2S/1 -> SOC_Mux/1  "SOC_cell1"
  SOC2_PS2S/1 -> SOC_Mux/2  "SOC_cell2"
  SOC3_PS2S/1 -> SOC_Mux/3  "SOC_cell3"
  SOC_Mux/1 -> Balancer/1, SOC_Scope/1
  BalEnable/1 -> Balancer/2
  Balancer/1 -> Bal_Scope/1, CmdDelay/1
  Cmd_Demux/1 -> Cmd1_S2PS/1
  Cmd_Demux/2 -> Cmd2_S2PS/1
  Cmd_Demux/3 -> Cmd3_S2PS/1
  Balancer/2 -> Bal_Scope/2
  CmdDelay/1 -> Cmd_Demux/1
  connections:
  Charger/LConn1 -- Isense/LConn1
  Rbleed2/RConn1 -- Vcell2/RConn2 -- Cell1/RConn1 -- Subsystem1/LConn4 -- BalSW1/LConn1 -- Vcell1/LConn1 -- Cell/LConn1
  Vcell1/RConn2 -- Rbleed1/RConn1 -- Cell/RConn1 -- Solver/RConn1 -- GND/LConn1 -- Charger/RConn2
  S2PS/RConn1 -- Charger/RConn1
  Subsystem1/LConn5 -- Vcell3/RConn2 -- Rbleed3/RConn1 -- Cell2/RConn1 -- Vcell2/LConn1 -- Cell1/LConn1 -- BalSW2/LConn1
  Subsystem1/LConn1 -- Isense/RConn1
  Subsystem1/LConn2 -- Cell/LConn2 -- SOC1_PS2S/LConn1
  Subsystem1/LConn3 -- Cell1/LConn2 -- SOC2_PS2S/LConn1
  GND1/LConn1 -- Subsystem1/RConn1
  Isense/RConn2 -- Subsystem1/LConn7 -- Cell2/LConn1 -- Vcell3/LConn1 -- BalSW3/LConn1
  Subsystem1/LConn6 -- Cell2/LConn2 -- SOC3_PS2S/LConn1
  Vcell1/RConn1 -- Vc1_PS2S/LConn1
  Vcell2/RConn1 -- Vc2_PS2S/LConn1
  Vcell3/RConn1 -- Vc3_PS2S/LConn1
  BalSW1/RConn2 -- Rbleed1/LConn1
  Cmd1_S2PS/RConn1 -- BalSW1/RConn1
  BalSW2/RConn2 -- Rbleed2/LConn1
  Cmd2_S2PS/RConn1 -- BalSW2/RConn1
  BalSW3/RConn2 -- Rbleed3/LConn1
  Cmd3_S2PS/RConn1 -- BalSW3/RConn1

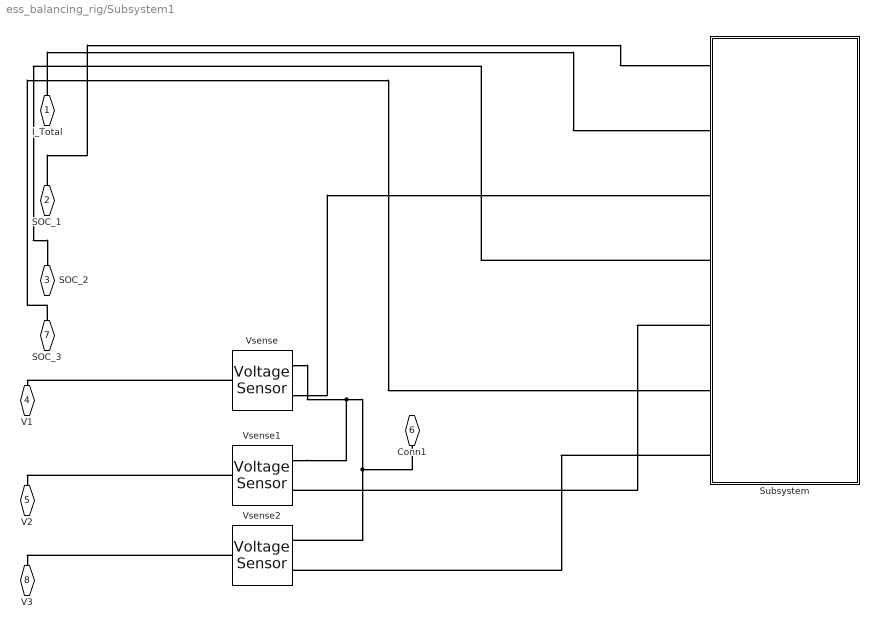
== system ess_balancing_rig/Subsystem1 ==
  Subsystem : Subsystem
  Vsense : fl_lib/Electrical/Electrical Sensors/Voltage Sensor
  Vsense1 : fl_lib/Electrical/Electrical Sensors/Voltage Sensor
  Vsense2 : fl_lib/Electrical/Electrical Sensors/Voltage Sensor
  I_Total : PMIOPort  Side=Left
  SOC_1 : PMIOPort  Port=2  Side=Left
  SOC_2 : PMIOPort  Port=3  Side=Left
  V1 : PMIOPort  Port=4  Side=Left
  V2 : PMIOPort  Port=5  Side=Left
  Conn1 : PMIOPort  Port=6  Side=Right
  SOC_3 : PMIOPort  Port=7  Side=Left
  V3 : PMIOPort  Port=8  Side=Left
  connections:
  SOC_1/RConn1 -- Subsystem/LConn1
  Subsystem/LConn5 -- Vsense1/RConn1
  Subsystem/LConn4 -- SOC_2/RConn1
  I_Total/RConn1 -- Subsystem/LConn2
  Vsense1/RConn2 -- Vsense2/RConn2 -- Conn1/RConn1 -- Vsense/RConn2
  Vsense/RConn1 -- Subsystem/LConn3
  Vsense1/LConn1 -- V2/RConn1
  Vsense/LConn1 -- V1/RConn1
  SOC_3/RConn1 -- Subsystem/LConn6
  Vsense2/LConn1 -- V3/RConn1
  Subsystem/LConn7 -- Vsense2/RConn1

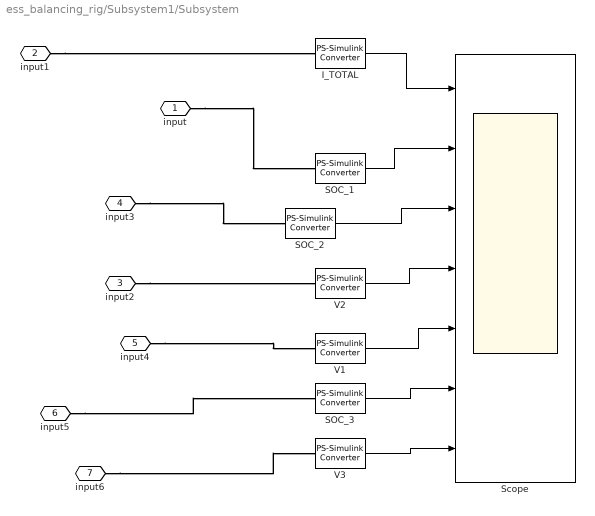
== system ess_balancing_rig/Subsystem1/Subsystem ==
  I_TOTAL : nesl_utility/PS-Simulink Converter  PhysicalDomain=network_engine_domain  SubClassName=ps_output  LeftPortType=input  RightPortType=output  PseudoPeriodic=off  Frequencies=[]  VectorFormat=inherit  Unit=inherit  AffineConversion=off
  SOC_1 : nesl_utility/PS-Simulink Converter  PhysicalDomain=network_engine_domain  SubClassName=ps_output  LeftPortType=input  RightPortType=output  PseudoPeriodic=off  Frequencies=[]  VectorFormat=inherit  Unit=inherit  AffineConversion=off
  SOC_2 : nesl_utility/PS-Simulink Converter  PhysicalDomain=network_engine_domain  SubClassName=ps_output  LeftPortType=input  RightPortType=output  PseudoPeriodic=off  Frequencies=[]  VectorFormat=inherit  Unit=inherit  AffineConversion=off
  SOC_3 : nesl_utility/PS-Simulink Converter  PhysicalDomain=network_engine_domain  SubClassName=ps_output  LeftPortType=input  RightPortType=output  PseudoPeriodic=off  Frequencies=[]  VectorFormat=inherit  Unit=inherit  AffineConversion=off
  Scope : Scope  NumInputPorts=7
      settings: ActiveDisplayYMinimum=-0.50581922809664936  ActiveDisplayYMaximum=1.6927751823037425  DataLoggingVariableName=scopeData
  V1 : nesl_utility/PS-Simulink Converter  PhysicalDomain=network_engine_domain  SubClassName=ps_output  LeftPortType=input  RightPortType=output  PseudoPeriodic=off  Frequencies=[]  VectorFormat=inherit  Unit=inherit  AffineConversion=off
  V2 : nesl_utility/PS-Simulink Converter  PhysicalDomain=network_engine_domain  SubClassName=ps_output  LeftPortType=input  RightPortType=output  PseudoPeriodic=off  Frequencies=[]  VectorFormat=inherit  Unit=inherit  AffineConversion=off
  V3 : nesl_utility/PS-Simulink Converter  PhysicalDomain=network_engine_domain  SubClassName=ps_output  LeftPortType=input  RightPortType=output  PseudoPeriodic=off  Frequencies=[]  VectorFormat=inherit  Unit=inherit  AffineConversion=off
  input : PMIOPort  Side=Left
  input1 : PMIOPort  Port=2  Side=Left
  input2 : PMIOPort  Port=3  Side=Left
  input3 : PMIOPort  Port=4  Side=Left
  input4 : PMIOPort  Port=5  Side=Left
  input5 : PMIOPort  Port=6  Side=Left
  input6 : PMIOPort  Port=7  Side=Left
  wires:
  SOC_1/1 -> Scope/2
  V2/1 -> Scope/4
  I_TOTAL/1 -> Scope/1
  SOC_2/1 -> Scope/3
  V1/1 -> Scope/5
  SOC_3/1 -> Scope/6
  V3/1 -> Scope/7
  connections:
  input1/RConn1 -- I_TOTAL/LConn1
  input2/RConn1 -- V2/LConn1
  input/RConn1 -- SOC_1/LConn1
  input3/RConn1 -- SOC_2/LConn1
  input4/RConn1 -- V1/LConn1
  input6/RConn1 -- V3/LConn1
  input5/RConn1 -- SOC_3/LConn1
